simulink model "sm_car"  (R2025a)
settings: Solver=ode23t  StartTime=0.0  StopTime=400  MaxStep=0.4  RelTol=1e-3  AbsTol=1e-3  EnableMultiTasking=on
PreLoadFcn:
  | % Due to usability issue in Repeating Sequence block
  | warning('off','Simulink:Masking:Invalid');
  | 
  | % Eliminate unnecessary warnings in inactive variants
  | % Warnings generated only if you click through inactive variant
  | warning('off','MATLAB:nonExistentField');
  | warning('off','Simulink:Parameters:BlkParamUndefined');
PostLoadFcn:
  | set_param([bdroot '/Vehicle'],'popup_trailer','Off')
  | warning('off','sm:sli:setup:compile:LocalSolverNotSupported')
  | %sm_car_config_maneuver(bdroot,'WOT Braking');
  | sm_car_config_vehicle(bdroot,'false');
  | sm_car_config_logging(bdroot);
InitFcn:
  | sm_car_config_camera;
  | Vehicle = sm_car_vehcfg_checkConfig(Vehicle);
  | sm_car_check_tire_model(bdroot);
StartFcn:
  | tic;
StopFcn:
  | Elapsed_Sim_Time = toc;
  | % disp(['Elapsed Sim Time = ' num2str(Elapsed_Sim_Time)]);
undefined symbols (not defined in the file): Axle1D, AxleIn, Camera, Control, Driver, Free, Init, Maneuver, Pedal, RaceFix, RaceSpin, Scene, ShaftL1, ShaftL2, ShaftR1, ShaftR2, Soft, Stiff, Visual, X, xy_data_car_side, Y, Z
libraries: sm_lib x1546, nesl_utility x528, fl_lib x480, SimscapeFluids_lib x61, sdl_lib x49, simulink x29, ee_lib x7, simulink_extras x6, Linkage_Systems x4, Tire_1x2x x4, AntiRollBar_Systems x2, Linkage_Decoupled x2
(part 16 of 79)

== system sm_car/Controller/TrqVec 4Motor/Brake Control/ABS/Valve Control L2/Subsystem ==
  OnT : Inport
  Constant : Constant  Value=0
  Constant1 : Constant
  Demux : Demux  Outputs=9
  Multiport Switch : MultiPortSwitch  DataPortOrder=Zero-based contiguous  Inputs=11  zeroidx=on  SaturateOnIntegerOverflow=off  InputSameDT=off
  Pulse Generator : DiscretePulseGenerator  PulseType=Time based  Period=0.01  PulseWidth=[1 2 3 4 5 6 7 8 9]*10
  vSig : Outport  VectorParamsAs1DForOutWhenUnconnected=off
  wires:
  Multiport Switch/1 -> vSig/1
  Demux/9 -> Multiport Switch/11
  Demux/8 -> Multiport Switch/10
  Demux/7 -> Multiport Switch/9
  Demux/6 -> Multiport Switch/8
  Demux/5 -> Multiport Switch/7
  Demux/4 -> Multiport Switch/6
  Demux/3 -> Multiport Switch/5
  Demux/2 -> Multiport Switch/4
  Demux/1 -> Multiport Switch/3
  OnT/1 -> Multiport Switch/1
  Constant1/1 -> Multiport Switch/12
  Constant/1 -> Multiport Switch/2
  Pulse Generator/1 -> Demux/1

== system sm_car/Controller/TrqVec 4Motor/Brake Control/ABS/Valve Control L2/Subsystem1 ==
  OnT : Inport
  Constant : Constant  Value=0
  Constant1 : Constant
  Demux : Demux  Outputs=9
  Multiport Switch : MultiPortSwitch  DataPortOrder=Zero-based contiguous  Inputs=11  zeroidx=on  SaturateOnIntegerOverflow=off  InputSameDT=off
  Pulse Generator : DiscretePulseGenerator  PulseType=Time based  Period=0.01  PulseWidth=[1 2 3 4 5 6 7 8 9]*10
  vSig : Outport  VectorParamsAs1DForOutWhenUnconnected=off
  wires:
  Pulse Generator/1 -> Demux/1
  Constant/1 -> Multiport Switch/2
  Constant1/1 -> Multiport Switch/12
  OnT/1 -> Multiport Switch/1
  Demux/1 -> Multiport Switch/3
  Demux/2 -> Multiport Switch/4
  Demux/3 -> Multiport Switch/5
  Demux/4 -> Multiport Switch/6
  Demux/5 -> Multiport Switch/7
  Demux/6 -> Multiport Switch/8
  Demux/7 -> Multiport Switch/9
  Demux/8 -> Multiport Switch/10
  Demux/9 -> Multiport Switch/11
  Multiport Switch/1 -> vSig/1

== system sm_car/Controller/TrqVec 4Motor/Brake Control/ABS/Valve Control R1/Categorize Surface ==
  Mod State : Inport
  Apply Valve : Inport  Port=2
  Compare To Constant : simulink/Logic and Bit Operations/Compare To Constant  relop=<  const=4  OutDataTypeStr=boolean
  Compare To Constant1 : simulink/Logic and Bit Operations/Compare To Constant  relop===  const=2  OutDataTypeStr=boolean
  Count Apply Pulses : Subsystem  TreatAsAtomicUnit=on
  Terminator : Terminator
  Total Apply Pulses This Cycle : Subsystem  TreatAsAtomicUnit=on
  wires:
  Compare To Constant/1 -> Terminator/1  "Low Mu"
  Total Apply Pulses This Cycle/1(Total Pulses) -> Compare To Constant/1
  Compare To Constant1/1 -> Count Apply Pulses/1(In1)
  Mod State/1 -> Compare To Constant1/1, Total Apply Pulses This Cycle/Trigger  "Transition to Release"
  Apply Valve/1 -> Count Apply Pulses/Trigger
  Count Apply Pulses/1(Apply Pulses) -> Total Apply Pulses This Cycle/1(In1)

== system sm_car/Controller/TrqVec 4Motor/Brake Control/ABS/Valve Control R1/Code to Valves ==
  note: Release
  note: Hold
  note: Apply
  C : Inport
  Constant : Constant  Value=[0 0]
  Constant1 : Constant  Value=[0 1]
  Constant2 : Constant  Value=[1 0]
  Multiport Switch : MultiPortSwitch  DataPortOrder=Zero-based contiguous  zeroidx=on  SaturateOnIntegerOverflow=off  InputSameDT=off
  V : Outport  VectorParamsAs1DForOutWhenUnconnected=off
  wires:
  Multiport Switch/1 -> V/1
  C/1 -> Multiport Switch/1
  Constant2/1 -> Multiport Switch/4
  Constant1/1 -> Multiport Switch/3
  Constant/1 -> Multiport Switch/2

== system sm_car/Controller/TrqVec 4Motor/Brake Control/ABS/Valve Control R1/Subsystem ==
  OnT : Inport
  Constant : Constant  Value=0
  Constant1 : Constant
  Demux : Demux  Outputs=9
  Multiport Switch : MultiPortSwitch  DataPortOrder=Zero-based contiguous  Inputs=11  zeroidx=on  SaturateOnIntegerOverflow=off  InputSameDT=off
  Pulse Generator : DiscretePulseGenerator  PulseType=Time based  Period=0.01  PulseWidth=[1 2 3 4 5 6 7 8 9]*10
  vSig : Outport  VectorParamsAs1DForOutWhenUnconnected=off
  wires:
  Multiport Switch/1 -> vSig/1
  Demux/9 -> Multiport Switch/11
  Demux/8 -> Multiport Switch/10
  Demux/7 -> Multiport Switch/9
  Demux/6 -> Multiport Switch/8
  Demux/5 -> Multiport Switch/7
  Demux/4 -> Multiport Switch/6
  Demux/3 -> Multiport Switch/5
  Demux/2 -> Multiport Switch/4
  Demux/1 -> Multiport Switch/3
  OnT/1 -> Multiport Switch/1
  Constant1/1 -> Multiport Switch/12
  Constant/1 -> Multiport Switch/2
  Pulse Generator/1 -> Demux/1

== system sm_car/Controller/TrqVec 4Motor/Brake Control/ABS/Valve Control R1/Subsystem1 ==
  OnT : Inport
  Constant : Constant  Value=0
  Constant1 : Constant
  Demux : Demux  Outputs=9
  Multiport Switch : MultiPortSwitch  DataPortOrder=Zero-based contiguous  Inputs=11  zeroidx=on  SaturateOnIntegerOverflow=off  InputSameDT=off
  Pulse Generator : DiscretePulseGenerator  PulseType=Time based  Period=0.01  PulseWidth=[1 2 3 4 5 6 7 8 9]*10
  vSig : Outport  VectorParamsAs1DForOutWhenUnconnected=off
  wires:
  Pulse Generator/1 -> Demux/1
  Constant/1 -> Multiport Switch/2
  Constant1/1 -> Multiport Switch/12
  OnT/1 -> Multiport Switch/1
  Demux/1 -> Multiport Switch/3
  Demux/2 -> Multiport Switch/4
  Demux/3 -> Multiport Switch/5
  Demux/4 -> Multiport Switch/6
  Demux/5 -> Multiport Switch/7
  Demux/6 -> Multiport Switch/8
  Demux/7 -> Multiport Switch/9
  Demux/8 -> Multiport Switch/10
  Demux/9 -> Multiport Switch/11
  Multiport Switch/1 -> vSig/1

== system sm_car/Controller/TrqVec 4Motor/Brake Control/ABS/Valve Control R2/Categorize Surface ==
  Mod State : Inport
  Apply Valve : Inport  Port=2
  Compare To Constant : simulink/Logic and Bit Operations/Compare To Constant  relop=<  const=4  OutDataTypeStr=boolean
  Compare To Constant1 : simulink/Logic and Bit Operations/Compare To Constant  relop===  const=2  OutDataTypeStr=boolean
  Count Apply Pulses : Subsystem  TreatAsAtomicUnit=on
  Terminator : Terminator
  Total Apply Pulses This Cycle : Subsystem  TreatAsAtomicUnit=on
  wires:
  Compare To Constant/1 -> Terminator/1  "Low Mu"
  Total Apply Pulses This Cycle/1(Total Pulses) -> Compare To Constant/1
  Compare To Constant1/1 -> Count Apply Pulses/1(In1)
  Mod State/1 -> Compare To Constant1/1, Total Apply Pulses This Cycle/Trigger  "Transition to Release"
  Apply Valve/1 -> Count Apply Pulses/Trigger
  Count Apply Pulses/1(Apply Pulses) -> Total Apply Pulses This Cycle/1(In1)

== system sm_car/Controller/TrqVec 4Motor/Brake Control/ABS/Valve Control R2/Code to Valves ==
  note: Release
  note: Hold
  note: Apply
  C : Inport
  Constant : Constant  Value=[0 0]
  Constant1 : Constant  Value=[0 1]
  Constant2 : Constant  Value=[1 0]
  Multiport Switch : MultiPortSwitch  DataPortOrder=Zero-based contiguous  zeroidx=on  SaturateOnIntegerOverflow=off  InputSameDT=off
  V : Outport  VectorParamsAs1DForOutWhenUnconnected=off
  wires:
  Multiport Switch/1 -> V/1
  C/1 -> Multiport Switch/1
  Constant2/1 -> Multiport Switch/4
  Constant1/1 -> Multiport Switch/3
  Constant/1 -> Multiport Switch/2

== system sm_car/Controller/TrqVec 4Motor/Brake Control/ABS/Valve Control R2/Subsystem ==
  OnT : Inport
  Constant : Constant  Value=0
  Constant1 : Constant
  Demux : Demux  Outputs=9
  Multiport Switch : MultiPortSwitch  DataPortOrder=Zero-based contiguous  Inputs=11  zeroidx=on  SaturateOnIntegerOverflow=off  InputSameDT=off
  Pulse Generator : DiscretePulseGenerator  PulseType=Time based  Period=0.01  PulseWidth=[1 2 3 4 5 6 7 8 9]*10
  vSig : Outport  VectorParamsAs1DForOutWhenUnconnected=off
  wires:
  Multiport Switch/1 -> vSig/1
  Demux/9 -> Multiport Switch/11
  Demux/8 -> Multiport Switch/10
  Demux/7 -> Multiport Switch/9
  Demux/6 -> Multiport Switch/8
  Demux/5 -> Multiport Switch/7
  Demux/4 -> Multiport Switch/6
  Demux/3 -> Multiport Switch/5
  Demux/2 -> Multiport Switch/4
  Demux/1 -> Multiport Switch/3
  OnT/1 -> Multiport Switch/1
  Constant1/1 -> Multiport Switch/12
  Constant/1 -> Multiport Switch/2
  Pulse Generator/1 -> Demux/1

== system sm_car/Controller/TrqVec 4Motor/Brake Control/ABS/Valve Control R2/Subsystem1 ==
  OnT : Inport
  Constant : Constant  Value=0
  Constant1 : Constant
  Demux : Demux  Outputs=9
  Multiport Switch : MultiPortSwitch  DataPortOrder=Zero-based contiguous  Inputs=11  zeroidx=on  SaturateOnIntegerOverflow=off  InputSameDT=off
  Pulse Generator : DiscretePulseGenerator  PulseType=Time based  Period=0.01  PulseWidth=[1 2 3 4 5 6 7 8 9]*10
  vSig : Outport  VectorParamsAs1DForOutWhenUnconnected=off
  wires:
  Pulse Generator/1 -> Demux/1
  Constant/1 -> Multiport Switch/2
  Constant1/1 -> Multiport Switch/12
  OnT/1 -> Multiport Switch/1
  Demux/1 -> Multiport Switch/3
  Demux/2 -> Multiport Switch/4
  Demux/3 -> Multiport Switch/5
  Demux/4 -> Multiport Switch/6
  Demux/5 -> Multiport Switch/7
  Demux/6 -> Multiport Switch/8
  Demux/7 -> Multiport Switch/9
  Demux/8 -> Multiport Switch/10
  Demux/9 -> Multiport Switch/11
  Multiport Switch/1 -> vSig/1

== system sm_car/Controller/TrqVec 4Motor/Damper Control/Damper Control A1/Coefficient/Filter ==
  In : Inport
  Gain : Gain  Gain=1/b
  Integrator : Integrator  InitialCondition=x_initial*b
  Sum : Sum  Inputs=|+-  InputSameDT=on  SaturateOnIntegerOverflow=on  OutDataTypeStr=Inherit: Same as first input
  Out : Outport  VectorParamsAs1DForOutWhenUnconnected=off
  wires:
  Sum/1 -> Integrator/1
  In/1 -> Sum/1
  Integrator/1 -> Gain/1
  Gain/1 -> Sum/2, Out/1

== system sm_car/Controller/TrqVec 4Motor/Damper Control/Damper Control A1/Force/Filter ==
  In : Inport
  Gain : Gain  Gain=1/b
  Integrator : Integrator  InitialCondition=x_initial*b
  Sum : Sum  Inputs=|+-  InputSameDT=on  SaturateOnIntegerOverflow=on  OutDataTypeStr=Inherit: Same as first input
  Out : Outport  VectorParamsAs1DForOutWhenUnconnected=off
  wires:
  Sum/1 -> Integrator/1
  In/1 -> Sum/1
  Integrator/1 -> Gain/1
  Gain/1 -> Sum/2, Out/1

== system sm_car/Controller/TrqVec 4Motor/Damper Control/Damper Control A2/Coefficient/Filter ==
  In : Inport
  Gain : Gain  Gain=1/b
  Integrator : Integrator  InitialCondition=x_initial*b
  Sum : Sum  Inputs=|+-  InputSameDT=on  SaturateOnIntegerOverflow=on  OutDataTypeStr=Inherit: Same as first input
  Out : Outport  VectorParamsAs1DForOutWhenUnconnected=off
  wires:
  Sum/1 -> Integrator/1
  In/1 -> Sum/1
  Integrator/1 -> Gain/1
  Gain/1 -> Sum/2, Out/1

== system sm_car/Controller/TrqVec 4Motor/Damper Control/Damper Control A2/Force/Filter ==
  In : Inport
  Gain : Gain  Gain=1/b
  Integrator : Integrator  InitialCondition=x_initial*b
  Sum : Sum  Inputs=|+-  InputSameDT=on  SaturateOnIntegerOverflow=on  OutDataTypeStr=Inherit: Same as first input
  Out : Outport  VectorParamsAs1DForOutWhenUnconnected=off
  wires:
  Sum/1 -> Integrator/1
  In/1 -> Sum/1
  Integrator/1 -> Gain/1
  Gain/1 -> Sum/2, Out/1

== system sm_car/Vehicle/Vehicle/Chassis/Aero/Subsystem/Actuator dynamics ==
  In : Inport
  Gain : Gain  Gain=1/b
  Integrator : Integrator  InitialCondition=x_initial*b
  Sum : Sum  Inputs=|+-  InputSameDT=on  SaturateOnIntegerOverflow=on  OutDataTypeStr=Inherit: Same as first input
  Out : Outport  VectorParamsAs1DForOutWhenUnconnected=off
  wires:
  Sum/1 -> Integrator/1
  In/1 -> Sum/1
  Integrator/1 -> Gain/1
  Gain/1 -> Sum/2, Out/1

== system sm_car/Vehicle/Vehicle/Chassis/Body/Body Geometry/CAD FSAE Achilles ==
  Aero : Subsystem
  Body : Subsystem
  Rollbar : sm_lib/Body Elements/File Solid  ExtGeomFileName=FSAE_Rollbar.STL  UnitType=Custom  ExtGeomFileUnits=m  StepReaderType=HEX  ExportConvexHullGeometry=off  InertiaType=PointMass  BasedOnType=Density  Density=700.769  DensityUnits=kg/m^3  Mass=0  MassUnits=kg  CenterOfMass=[0.988684, 1.00464/1.8, 2.92072]  CenterOfMassUnits=m  MomentsOfInertia=[478.463, 518.088, 108.52]  MomentsOfInertiaUnits=kg*m^2  ProductsOfInertia=[-18.6469, 0.0347848, 0.00267861]  ProductsOfInertiaUnits=kg*m^2  GraphicType=FromGeometry  MarkerShape=Sphere  MarkerSize=10  GraphicVisPropType=SimpleVisualProperties  GraphicDiffuseColor=[0.6 0.6 0.6]  GraphicOpacity=1  GraphicSpecularColor=[0.5 0.5 0.5 1.0]  GraphicAmbientColor=[0.15 0.15 0.15 1.0]  GraphicEmissiveColor=[0.0 0.0 0.0 1.0]  GraphicShininess=75  DoExposeReferenceFrame=on  SerializedFrames=<Frames/>
  Seat : sm_lib/Body Elements/File Solid  ExtGeomFileName=FSAE_Seat.STL  UnitType=Custom  ExtGeomFileUnits=m  StepReaderType=HEX  ExportConvexHullGeometry=off  InertiaType=PointMass  BasedOnType=Density  Density=700.769  DensityUnits=kg/m^3  Mass=0  MassUnits=kg  CenterOfMass=[0.988684, 1.00464/1.8, 2.92072]  CenterOfMassUnits=m  MomentsOfInertia=[478.463, 518.088, 108.52]  MomentsOfInertiaUnits=kg*m^2  ProductsOfInertia=[-18.6469, 0.0347848, 0.00267861]  ProductsOfInertiaUnits=kg*m^2  GraphicType=FromGeometry  MarkerShape=Sphere  MarkerSize=10  GraphicVisPropType=SimpleVisualProperties  GraphicDiffuseColor=[0.2 0.2 0.2]  GraphicOpacity=1  GraphicSpecularColor=[0.5 0.5 0.5 1.0]  GraphicAmbientColor=[0.15 0.15 0.15 1.0]  GraphicEmissiveColor=[0.0 0.0 0.0 1.0]  GraphicShininess=75  DoExposeReferenceFrame=on  SerializedFrames=<Frames/>
  Transform CAD Offset : sm_lib/Frames and Transforms/Rigid Transform  RotationMethod=RotationSequence  FollAlignAxisA=+Y  BaseAlignAxisA=+Z  FollAlignAxisB=-X  BaseAlignAxisB=+Y  RotationStandardAxis=+Z  RotationAngle=0  RotationAngleUnits=deg  RotationArbitraryAxis=[0 0 1]  RotationSequenceAxes=FollowerAxes  RotationSequence=ZYX  RotationSequenceAngles=[body_orient(3) body_orient(2) body_orient(1)]  RotationSequenceAnglesUnits=rad  RotationMatrix=[1 0 0; 0 1 0; 0 0 1]  Quaternion=[1 0 0 0]  TranslationMethod=Cartesian  TranslationCartesianOffset=body_offset  TranslationCartesianOffsetUnits=m  TranslationStandardAxis=+Z  TranslationStandardOffset=0  TranslationStandardOffsetUnits=m  TranslationROffset=0  TranslationROffsetUnits=m  TranslationThetaOffset=0  TranslationThetaOffsetUnits=deg  TranslationZOffset=0  TranslationZOffsetUnits=m
  FA : PMIOPort  Side=Right
  P : PMIOPort  Port=2  Side=Left
  connections:
  Aero/RConn1 -- Transform CAD Offset/RConn1 -- Seat/RConn1 -- Body/LConn1 -- Rollbar/RConn1
  FA/RConn1 -- P/RConn1 -- Transform CAD Offset/LConn1

== system sm_car/Vehicle/Vehicle/Chassis/Body/Body Load/None ==
  FA : PMIOPort  Side=Left

== system sm_car/Vehicle/Vehicle/Chassis/Body/Body Sensor/Roll Pitch ==
  R : Inport
  Calculate aPitch : Subsystem
  Calculate aRoll : Subsystem
  "Flip sign for -x axis " : Gain  Gain=-1
  Select x axis : Selector  NumberOfDimensions=2  InputPortWidth=2  IndexOptions=Index vector (dialog),Index vector (dialog)  Indices=[1 2 3],1  OutputSizes=1,1
  Select y axis : Selector  NumberOfDimensions=2  InputPortWidth=2  IndexOptions=Index vector (dialog),Index vector (dialog)  Indices=[1 2 3],2  OutputSizes=1,1
  Transfer Fcn : TransferFcn  Numerator=[1 0]  Denominator=[0.01 1]
  Transfer Fcn1 : TransferFcn  Numerator=[1 0]  Denominator=[0.01 1]
  aRoll : Outport  VectorParamsAs1DForOutWhenUnconnected=off
  aPitch : Outport  Port=2  VectorParamsAs1DForOutWhenUnconnected=off
  nRoll : Outport  Port=3  VectorParamsAs1DForOutWhenUnconnected=off
  nPitch : Outport  Port=4  VectorParamsAs1DForOutWhenUnconnected=off
  wires:
  Calculate aPitch/1(Angle) -> "Flip sign for -x axis "/1
  Select x axis/1 -> Calculate aPitch/2(uvec)
  R/1 -> Select y axis/1, Select x axis/1
  Select y axis/1 -> Calculate aRoll/1(uvec)
  "Flip sign for -x axis "/1 -> aPitch/1, Transfer Fcn1/1
  Calculate aRoll/1(Angle) -> Transfer Fcn/1, aRoll/1, Calculate aPitch/1(Roll Angle)
  Transfer Fcn/1 -> nRoll/1
  Transfer Fcn1/1 -> nPitch/1

== system sm_car/Vehicle/Vehicle/Chassis/Body/Passenger FL/None ==
  Body Sensor Empty : Subsystem  mask{offset_body_sensor=Vehicle.Chassis.Body.sCG.Value}
      mask prompts: offset_body_sensor "Sensor Frame Offset [x y z] (m)"
  P : PMIOPort  Side=Left
  m : Outport  VectorParamsAs1DForOutWhenUnconnected=off
  wires:
  Body Sensor Empty/1(Body) -> m/1
  connections:
  Body Sensor Empty/LConn1 -- P/RConn1

== system sm_car/Vehicle/Vehicle/Chassis/Body/Passenger FR/None ==
  Body Sensor Empty : Subsystem  mask{offset_body_sensor=Vehicle.Chassis.Body.sCG.Value}
      mask prompts: offset_body_sensor "Sensor Frame Offset [x y z] (m)"
  P : PMIOPort  Side=Left
  m : Outport  VectorParamsAs1DForOutWhenUnconnected=off
  wires:
  Body Sensor Empty/1(Body) -> m/1
  connections:
  Body Sensor Empty/LConn1 -- P/RConn1

== system sm_car/Vehicle/Vehicle/Chassis/Body/Passenger RL/None ==
  Body Sensor Empty : Subsystem  mask{offset_body_sensor=Vehicle.Chassis.Body.sCG.Value}
      mask prompts: offset_body_sensor "Sensor Frame Offset [x y z] (m)"
  P : PMIOPort  Side=Left
  m : Outport  VectorParamsAs1DForOutWhenUnconnected=off
  wires:
  Body Sensor Empty/1(Body) -> m/1
  connections:
  Body Sensor Empty/LConn1 -- P/RConn1

== system sm_car/Vehicle/Vehicle/Chassis/Body/Passenger RR/None ==
  Body Sensor Empty : Subsystem  mask{offset_body_sensor=Vehicle.Chassis.Body.sCG.Value}
      mask prompts: offset_body_sensor "Sensor Frame Offset [x y z] (m)"
  P : PMIOPort  Side=Left
  m : Outport  VectorParamsAs1DForOutWhenUnconnected=off
  wires:
  Body Sensor Empty/1(Body) -> m/1
  connections:
  Body Sensor Empty/LConn1 -- P/RConn1

== system sm_car/Vehicle/Vehicle/Chassis/Damper/Decoupled/Damper A1 Heave ==
  "Ctrl " : Inport
  Force Endstop NL : Subsystem  VariantControl=Force_EndstopNL  mask(Variable Damping Force with Nonlinear Endstop){hp_dpr_top=Damper.Damping.sTop.Value, hp_dpr_bot=Damper.Damping.sBottom.Value, xEndstop=Damper.Endstop.xEndstop.Value, fEndstop=Damper.Endstop.fEndstop.Value}
      mask prompts: hp_dpr_top "HP Damper Top [xyz] (m)"; hp_dpr_bot "HP Damper Bottom [xyz] (m)"; xEndstop "Endstop Deformation Vector (m)"; fEndstop "Endstop Force Vector (m)"
      mask help: Variable damping force with a nonlinear endstop at top and bottom. The damping force is set using an input signal.
      mask init:
      | dam_x0 = norm(hp_dpr_top - hp_dpr_bot);
  Linear : Subsystem  VariantControl=Linear  mask(Linear Damper with Bumpstop){dam_b=Damper.Damping.d.Value, hp_dpr_top=Damper.Damping.sTop.Value, hp_dpr_bot=Damper.Damping.sBottom.Value, bs_lim_upper=Damper.Endstop.xMax.Value, bs_lim_lower=Damper.Endstop.xMin.Value, bs_k_upper=Damper.Endstop.KxMax.Value, bs_k_lower=Damper.Endstop.KxMin.Value, bs_b_upper=Damper.Endstop.dxMax.Value, bs_b_lower=Damper.Endstop.dxMin.Value, bs_region=Damper.Endstop.xTransition.Value}
      mask prompts: dam_b "Damper (N/(m/s))"; hp_dpr_top "HP Damper Top [xyz] (m)"; hp_dpr_bot "HP Damper Bottom [xyz] (m)"; bs_region "Transition Region (m)"
      mask help: Linear damper with bumpstop at top and bottom.
      mask init:
      | dam_x0 = norm(hp_dpr_top - hp_dpr_bot);
      mask TypeOptions dam_b: Damper/D
      mask DialogControl text_bumpstop_upper Prompt: Upper
      mask DialogControl text_bumpstop_lower Prompt: Lower
      mask DialogControl text_bumpstop_limit Prompt: Limit (m)
      mask DialogControl text_bumpstop_k Prompt: Stiffness (N/m)
      mask DialogControl text_bumpstop_b Prompt: Damping  (N/(m/s))
  None : Subsystem  VariantControl=None  mask(No Damper){}
      mask help: Sensor only
  Nonlinear : Subsystem  VariantControl=Nonlinear  mask(Nonlinear Damper with Bumpstop){velocity_vector=Damper.Damping.vDamper.Value, force_vector=Damper.Damping.fDamper.Value, hp_dpr_top=Damper.Damping.sTop.Value, hp_dpr_bot=Damper.Damping.sBottom.Value, bs_lim_upper=Damper.Endstop.xMax.Value, bs_lim_lower=Damper.Endstop.xMin.Value, bs_k_upper=Damper.Endstop.KxMax.Value, bs_k_lower=Damper.Endstop.KxMin.Value, bs_b_upper=Damper.Endstop.dxMax.Value, bs_b_lower=Damper.Endstop.dxMin.Value, bs_region=Damper.Endstop.xTransition.Value}
      mask prompts: velocity_vector "Velocity vector"; force_vector "Force vector"; hp_dpr_top "HP Damper Top [xyz] (m)"; hp_dpr_bot "HP Damper Bottom [xyz] (m)"; bs_region "Transition Region (m)"
      mask help: Damper with damping coefficient specified as a lookup table in parallel with a bumpstop.
      mask init:
      | dam_x0 = norm(hp_dpr_top - hp_dpr_bot);
      mask TypeOptions velocity_vector: Damper/velocity_vector
      mask TypeOptions force_vector: Damper/force_vector
      mask DialogControl text_bumpstop_upper Prompt: Upper
      mask DialogControl text_bumpstop_lower Prompt: Lower
      mask DialogControl text_bumpstop_limit Prompt: Limit (m)
      mask DialogControl text_bumpstop_k Prompt: Stiffness (N/m)
      mask DialogControl text_bumpstop_b Prompt: Damping  (N/(m/s))
  Nonlinear Endstop NL : Subsystem  VariantControl=Nonlinear_EndstopNL  mask(Nonlinear Damper with Nonlinear Bumpstop){velocity_vector=Damper.Damping.vDamper.Value, force_vector=Damper.Damping.fDamper.Value, hp_dpr_top=Damper.Damping.sTop.Value, hp_dpr_bot=Damper.Damping.sBottom.Value, xEndstop=Damper.Endstop.xEndstop.Value, fEndstop=Damper.Endstop.fEndstop.Value}
      mask prompts: velocity_vector "Velocity vector"; force_vector "Force vector"; hp_dpr_top "HP Damper Top [xyz] (m)"; hp_dpr_bot "HP Damper Bottom [xyz] (m)"; xEndstop "Endstop Deformation Vector (m)"; fEndstop "Endstop Force Vector (m)"
      mask help: Damper with damping coefficient specified as a lookup table in parallel with a nonlinear endstop at top and bottom.
      mask init:
      | dam_x0 = norm(hp_dpr_top - hp_dpr_bot);
      mask TypeOptions velocity_vector: Damper/velocity_vector
      mask TypeOptions force_vector: Damper/force_vector
      mask TypeOptions xEndstop: Bumpstop/deformation_vector
      mask TypeOptions fEndstop: Bumpstop/force_vector
  Variable : Subsystem  VariantControl=Variable  mask(Variable Damper with Endstop){hp_dpr_top=Damper.Damping.sTop.Value, hp_dpr_bot=Damper.Damping.sBottom.Value, bs_lim_upper=Damper.Endstop.xMax.Value, bs_lim_lower=Damper.Endstop.xMin.Value, bs_k_upper=Damper.Endstop.KxMax.Value, bs_k_lower=Damper.Endstop.KxMin.Value, bs_b_upper=Damper.Endstop.dxMax.Value, bs_b_lower=Damper.Endstop.dxMin.Value, bs_region=Damper.Endstop.xTransition.Value}
      mask prompts: hp_dpr_top "HP Damper Top [xyz] (m)"; hp_dpr_bot "HP Damper Bottom [xyz] (m)"; bs_region "Transition Region (m)"
      mask help: Variable damper with endstop at top and bottom. The damping coefficient is set using an input signal.
      mask init:
      | dam_x0 = norm(hp_dpr_top - hp_dpr_bot);
      mask DialogControl text_bumpstop_upper Prompt: Upper
      mask DialogControl text_bumpstop_lower Prompt: Lower
      mask DialogControl text_bumpstop_limit Prompt: Limit (m)
      mask DialogControl text_bumpstop_k Prompt: Stiffness (N/m)
      mask DialogControl text_bumpstop_b Prompt: Damping  (N/(m/s))
  Variable Endstop NL : Subsystem  VariantControl=Variable_EndstopNL  mask(Variable Damper with Nonlinear Endstop){hp_dpr_top=Damper.Damping.sTop.Value, hp_dpr_bot=Damper.Damping.sBottom.Value, xEndstop=Damper.Endstop.xEndstop.Value, fEndstop=Damper.Endstop.fEndstop.Value}
      mask prompts: hp_dpr_top "HP Damper Top [xyz] (m)"; hp_dpr_bot "HP Damper Bottom [xyz] (m)"; xEndstop "Endstop Deformation Vector (m)"; fEndstop "Endstop Force Vector (m)"
      mask help: Variable damper with nonlinear endstop at top and bottom. The damping coefficient is set using an input signal.
      mask init:
      | dam_x0 = norm(hp_dpr_top - hp_dpr_bot);
  " R" : PMIOPort  Side=Left
  " C" : PMIOPort  Port=2  Side=Right
  " meas" : Outport  VectorParamsAs1DForOutWhenUnconnected=off

== system sm_car/Vehicle/Vehicle/Chassis/Damper/Decoupled/Damper A1 Roll ==
  "Ctrl " : Inport
  Force Endstop NL : Subsystem  VariantControl=Force_EndstopNL  mask(Variable Damping Force with Nonlinear Endstop){hp_dpr_top=Damper.Damping.sTop.Value, hp_dpr_bot=Damper.Damping.sBottom.Value, xEndstop=Damper.Endstop.xEndstop.Value, fEndstop=Damper.Endstop.fEndstop.Value}
      mask prompts: hp_dpr_top "HP Damper Top [xyz] (m)"; hp_dpr_bot "HP Damper Bottom [xyz] (m)"; xEndstop "Endstop Deformation Vector (m)"; fEndstop "Endstop Force Vector (m)"
      mask help: Variable damping force with a nonlinear endstop at top and bottom. The damping force is set using an input signal.
      mask init:
      | dam_x0 = norm(hp_dpr_top - hp_dpr_bot);
  Linear : Subsystem  VariantControl=Linear  mask(Linear Damper with Bumpstop){dam_b=Damper.Damping.d.Value, hp_dpr_top=Damper.Damping.sTop.Value, hp_dpr_bot=Damper.Damping.sBottom.Value, bs_lim_upper=Damper.Endstop.xMax.Value, bs_lim_lower=Damper.Endstop.xMin.Value, bs_k_upper=Damper.Endstop.KxMax.Value, bs_k_lower=Damper.Endstop.KxMin.Value, bs_b_upper=Damper.Endstop.dxMax.Value, bs_b_lower=Damper.Endstop.dxMin.Value, bs_region=Damper.Endstop.xTransition.Value}
      mask prompts: dam_b "Damper (N/(m/s))"; hp_dpr_top "HP Damper Top [xyz] (m)"; hp_dpr_bot "HP Damper Bottom [xyz] (m)"; bs_region "Transition Region (m)"
      mask help: Linear damper with bumpstop at top and bottom.
      mask init:
      | dam_x0 = norm(hp_dpr_top - hp_dpr_bot);
      mask TypeOptions dam_b: Damper/D
      mask DialogControl text_bumpstop_upper Prompt: Upper
      mask DialogControl text_bumpstop_lower Prompt: Lower
      mask DialogControl text_bumpstop_limit Prompt: Limit (m)
      mask DialogControl text_bumpstop_k Prompt: Stiffness (N/m)
      mask DialogControl text_bumpstop_b Prompt: Damping  (N/(m/s))
  None : Subsystem  VariantControl=None  mask(No Damper){}
      mask help: Sensor only
  Nonlinear : Subsystem  VariantControl=Nonlinear  mask(Nonlinear Damper with Bumpstop){velocity_vector=Damper.Damping.vDamper.Value, force_vector=Damper.Damping.fDamper.Value, hp_dpr_top=Damper.Damping.sTop.Value, hp_dpr_bot=Damper.Damping.sBottom.Value, bs_lim_upper=Damper.Endstop.xMax.Value, bs_lim_lower=Damper.Endstop.xMin.Value, bs_k_upper=Damper.Endstop.KxMax.Value, bs_k_lower=Damper.Endstop.KxMin.Value, bs_b_upper=Damper.Endstop.dxMax.Value, bs_b_lower=Damper.Endstop.dxMin.Value, bs_region=Damper.Endstop.xTransition.Value}
      mask prompts: velocity_vector "Velocity vector"; force_vector "Force vector"; hp_dpr_top "HP Damper Top [xyz] (m)"; hp_dpr_bot "HP Damper Bottom [xyz] (m)"; bs_region "Transition Region (m)"
      mask help: Damper with damping coefficient specified as a lookup table in parallel with a bumpstop.
      mask init:
      | dam_x0 = norm(hp_dpr_top - hp_dpr_bot);
      mask TypeOptions velocity_vector: Damper/velocity_vector
      mask TypeOptions force_vector: Damper/force_vector
      mask DialogControl text_bumpstop_upper Prompt: Upper
      mask DialogControl text_bumpstop_lower Prompt: Lower
      mask DialogControl text_bumpstop_limit Prompt: Limit (m)
      mask DialogControl text_bumpstop_k Prompt: Stiffness (N/m)
      mask DialogControl text_bumpstop_b Prompt: Damping  (N/(m/s))
  Nonlinear Endstop NL : Subsystem  VariantControl=Nonlinear_EndstopNL  mask(Nonlinear Damper with Nonlinear Bumpstop){velocity_vector=Damper.Damping.vDamper.Value, force_vector=Damper.Damping.fDamper.Value, hp_dpr_top=Damper.Damping.sTop.Value, hp_dpr_bot=Damper.Damping.sBottom.Value, xEndstop=Damper.Endstop.xEndstop.Value, fEndstop=Damper.Endstop.fEndstop.Value}
      mask prompts: velocity_vector "Velocity vector"; force_vector "Force vector"; hp_dpr_top "HP Damper Top [xyz] (m)"; hp_dpr_bot "HP Damper Bottom [xyz] (m)"; xEndstop "Endstop Deformation Vector (m)"; fEndstop "Endstop Force Vector (m)"
      mask help: Damper with damping coefficient specified as a lookup table in parallel with a nonlinear endstop at top and bottom.
      mask init:
      | dam_x0 = norm(hp_dpr_top - hp_dpr_bot);
      mask TypeOptions velocity_vector: Damper/velocity_vector
      mask TypeOptions force_vector: Damper/force_vector
      mask TypeOptions xEndstop: Bumpstop/deformation_vector
      mask TypeOptions fEndstop: Bumpstop/force_vector
  Variable : Subsystem  VariantControl=Variable  mask(Variable Damper with Endstop){hp_dpr_top=Damper.Damping.sTop.Value, hp_dpr_bot=Damper.Damping.sBottom.Value, bs_lim_upper=Damper.Endstop.xMax.Value, bs_lim_lower=Damper.Endstop.xMin.Value, bs_k_upper=Damper.Endstop.KxMax.Value, bs_k_lower=Damper.Endstop.KxMin.Value, bs_b_upper=Damper.Endstop.dxMax.Value, bs_b_lower=Damper.Endstop.dxMin.Value, bs_region=Damper.Endstop.xTransition.Value}
      mask prompts: hp_dpr_top "HP Damper Top [xyz] (m)"; hp_dpr_bot "HP Damper Bottom [xyz] (m)"; bs_region "Transition Region (m)"
      mask help: Variable damper with endstop at top and bottom. The damping coefficient is set using an input signal.
      mask init:
      | dam_x0 = norm(hp_dpr_top - hp_dpr_bot);
      mask DialogControl text_bumpstop_upper Prompt: Upper
      mask DialogControl text_bumpstop_lower Prompt: Lower
      mask DialogControl text_bumpstop_limit Prompt: Limit (m)
      mask DialogControl text_bumpstop_k Prompt: Stiffness (N/m)
      mask DialogControl text_bumpstop_b Prompt: Damping  (N/(m/s))
  Variable Endstop NL : Subsystem  VariantControl=Variable_EndstopNL  mask(Variable Damper with Nonlinear Endstop){hp_dpr_top=Damper.Damping.sTop.Value, hp_dpr_bot=Damper.Damping.sBottom.Value, xEndstop=Damper.Endstop.xEndstop.Value, fEndstop=Damper.Endstop.fEndstop.Value}
      mask prompts: hp_dpr_top "HP Damper Top [xyz] (m)"; hp_dpr_bot "HP Damper Bottom [xyz] (m)"; xEndstop "Endstop Deformation Vector (m)"; fEndstop "Endstop Force Vector (m)"
      mask help: Variable damper with nonlinear endstop at top and bottom. The damping coefficient is set using an input signal.
      mask init:
      | dam_x0 = norm(hp_dpr_top - hp_dpr_bot);
  " R" : PMIOPort  Side=Left
  " C" : PMIOPort  Port=2  Side=Right
  " meas" : Outport  VectorParamsAs1DForOutWhenUnconnected=off

== system sm_car/Vehicle/Vehicle/Chassis/Damper/Decoupled/Damper A2 Heave ==
  "Ctrl " : Inport
  Force Endstop NL : Subsystem  VariantControl=Force_EndstopNL  mask(Variable Damping Force with Nonlinear Endstop){hp_dpr_top=Damper.Damping.sTop.Value, hp_dpr_bot=Damper.Damping.sBottom.Value, xEndstop=Damper.Endstop.xEndstop.Value, fEndstop=Damper.Endstop.fEndstop.Value}
      mask prompts: hp_dpr_top "HP Damper Top [xyz] (m)"; hp_dpr_bot "HP Damper Bottom [xyz] (m)"; xEndstop "Endstop Deformation Vector (m)"; fEndstop "Endstop Force Vector (m)"
      mask help: Variable damping force with a nonlinear endstop at top and bottom. The damping force is set using an input signal.
      mask init:
      | dam_x0 = norm(hp_dpr_top - hp_dpr_bot);
  Linear : Subsystem  VariantControl=Linear  mask(Linear Damper with Bumpstop){dam_b=Damper.Damping.d.Value, hp_dpr_top=Damper.Damping.sTop.Value, hp_dpr_bot=Damper.Damping.sBottom.Value, bs_lim_upper=Damper.Endstop.xMax.Value, bs_lim_lower=Damper.Endstop.xMin.Value, bs_k_upper=Damper.Endstop.KxMax.Value, bs_k_lower=Damper.Endstop.KxMin.Value, bs_b_upper=Damper.Endstop.dxMax.Value, bs_b_lower=Damper.Endstop.dxMin.Value, bs_region=Damper.Endstop.xTransition.Value}
      mask prompts: dam_b "Damper (N/(m/s))"; hp_dpr_top "HP Damper Top [xyz] (m)"; hp_dpr_bot "HP Damper Bottom [xyz] (m)"; bs_region "Transition Region (m)"
      mask help: Linear damper with bumpstop at top and bottom.
      mask init:
      | dam_x0 = norm(hp_dpr_top - hp_dpr_bot);
      mask TypeOptions dam_b: Damper/D
      mask DialogControl text_bumpstop_upper Prompt: Upper
      mask DialogControl text_bumpstop_lower Prompt: Lower
      mask DialogControl text_bumpstop_limit Prompt: Limit (m)
      mask DialogControl text_bumpstop_k Prompt: Stiffness (N/m)
      mask DialogControl text_bumpstop_b Prompt: Damping  (N/(m/s))
  None : Subsystem  VariantControl=None  mask(No Damper){}
      mask help: Sensor only
  Nonlinear : Subsystem  VariantControl=Nonlinear  mask(Nonlinear Damper with Bumpstop){velocity_vector=Damper.Damping.vDamper.Value, force_vector=Damper.Damping.fDamper.Value, hp_dpr_top=Damper.Damping.sTop.Value, hp_dpr_bot=Damper.Damping.sBottom.Value, bs_lim_upper=Damper.Endstop.xMax.Value, bs_lim_lower=Damper.Endstop.xMin.Value, bs_k_upper=Damper.Endstop.KxMax.Value, bs_k_lower=Damper.Endstop.KxMin.Value, bs_b_upper=Damper.Endstop.dxMax.Value, bs_b_lower=Damper.Endstop.dxMin.Value, bs_region=Damper.Endstop.xTransition.Value}
      mask prompts: velocity_vector "Velocity vector"; force_vector "Force vector"; hp_dpr_top "HP Damper Top [xyz] (m)"; hp_dpr_bot "HP Damper Bottom [xyz] (m)"; bs_region "Transition Region (m)"
      mask help: Damper with damping coefficient specified as a lookup table in parallel with a bumpstop.
      mask init:
      | dam_x0 = norm(hp_dpr_top - hp_dpr_bot);
      mask TypeOptions velocity_vector: Damper/velocity_vector
      mask TypeOptions force_vector: Damper/force_vector
      mask DialogControl text_bumpstop_upper Prompt: Upper
      mask DialogControl text_bumpstop_lower Prompt: Lower
      mask DialogControl text_bumpstop_limit Prompt: Limit (m)
      mask DialogControl text_bumpstop_k Prompt: Stiffness (N/m)
      mask DialogControl text_bumpstop_b Prompt: Damping  (N/(m/s))
  Nonlinear Endstop NL : Subsystem  VariantControl=Nonlinear_EndstopNL  mask(Nonlinear Damper with Nonlinear Bumpstop){velocity_vector=Damper.Damping.vDamper.Value, force_vector=Damper.Damping.fDamper.Value, hp_dpr_top=Damper.Damping.sTop.Value, hp_dpr_bot=Damper.Damping.sBottom.Value, xEndstop=Damper.Endstop.xEndstop.Value, fEndstop=Damper.Endstop.fEndstop.Value}
      mask prompts: velocity_vector "Velocity vector"; force_vector "Force vector"; hp_dpr_top "HP Damper Top [xyz] (m)"; hp_dpr_bot "HP Damper Bottom [xyz] (m)"; xEndstop "Endstop Deformation Vector (m)"; fEndstop "Endstop Force Vector (m)"
      mask help: Damper with damping coefficient specified as a lookup table in parallel with a nonlinear endstop at top and bottom.
      mask init:
      | dam_x0 = norm(hp_dpr_top - hp_dpr_bot);
      mask TypeOptions velocity_vector: Damper/velocity_vector
      mask TypeOptions force_vector: Damper/force_vector
      mask TypeOptions xEndstop: Bumpstop/deformation_vector
      mask TypeOptions fEndstop: Bumpstop/force_vector
  Variable : Subsystem  VariantControl=Variable  mask(Variable Damper with Endstop){hp_dpr_top=Damper.Damping.sTop.Value, hp_dpr_bot=Damper.Damping.sBottom.Value, bs_lim_upper=Damper.Endstop.xMax.Value, bs_lim_lower=Damper.Endstop.xMin.Value, bs_k_upper=Damper.Endstop.KxMax.Value, bs_k_lower=Damper.Endstop.KxMin.Value, bs_b_upper=Damper.Endstop.dxMax.Value, bs_b_lower=Damper.Endstop.dxMin.Value, bs_region=Damper.Endstop.xTransition.Value}
      mask prompts: hp_dpr_top "HP Damper Top [xyz] (m)"; hp_dpr_bot "HP Damper Bottom [xyz] (m)"; bs_region "Transition Region (m)"
      mask help: Variable damper with endstop at top and bottom. The damping coefficient is set using an input signal.
      mask init:
      | dam_x0 = norm(hp_dpr_top - hp_dpr_bot);
      mask DialogControl text_bumpstop_upper Prompt: Upper
      mask DialogControl text_bumpstop_lower Prompt: Lower
      mask DialogControl text_bumpstop_limit Prompt: Limit (m)
      mask DialogControl text_bumpstop_k Prompt: Stiffness (N/m)
      mask DialogControl text_bumpstop_b Prompt: Damping  (N/(m/s))
  Variable Endstop NL : Subsystem  VariantControl=Variable_EndstopNL  mask(Variable Damper with Nonlinear Endstop){hp_dpr_top=Damper.Damping.sTop.Value, hp_dpr_bot=Damper.Damping.sBottom.Value, xEndstop=Damper.Endstop.xEndstop.Value, fEndstop=Damper.Endstop.fEndstop.Value}
      mask prompts: hp_dpr_top "HP Damper Top [xyz] (m)"; hp_dpr_bot "HP Damper Bottom [xyz] (m)"; xEndstop "Endstop Deformation Vector (m)"; fEndstop "Endstop Force Vector (m)"
      mask help: Variable damper with nonlinear endstop at top and bottom. The damping coefficient is set using an input signal.
      mask init:
      | dam_x0 = norm(hp_dpr_top - hp_dpr_bot);
  " R" : PMIOPort  Side=Left
  " C" : PMIOPort  Port=2  Side=Right
  " meas" : Outport  VectorParamsAs1DForOutWhenUnconnected=off

== system sm_car/Vehicle/Vehicle/Chassis/Damper/Decoupled/Damper A2 Roll ==
  "Ctrl " : Inport
  Force Endstop NL : Subsystem  VariantControl=Force_EndstopNL  mask(Variable Damping Force with Nonlinear Endstop){hp_dpr_top=Damper.Damping.sTop.Value, hp_dpr_bot=Damper.Damping.sBottom.Value, xEndstop=Damper.Endstop.xEndstop.Value, fEndstop=Damper.Endstop.fEndstop.Value}
      mask prompts: hp_dpr_top "HP Damper Top [xyz] (m)"; hp_dpr_bot "HP Damper Bottom [xyz] (m)"; xEndstop "Endstop Deformation Vector (m)"; fEndstop "Endstop Force Vector (m)"
      mask help: Variable damping force with a nonlinear endstop at top and bottom. The damping force is set using an input signal.
      mask init:
      | dam_x0 = norm(hp_dpr_top - hp_dpr_bot);
  Linear : Subsystem  VariantControl=Linear  mask(Linear Damper with Bumpstop){dam_b=Damper.Damping.d.Value, hp_dpr_top=Damper.Damping.sTop.Value, hp_dpr_bot=Damper.Damping.sBottom.Value, bs_lim_upper=Damper.Endstop.xMax.Value, bs_lim_lower=Damper.Endstop.xMin.Value, bs_k_upper=Damper.Endstop.KxMax.Value, bs_k_lower=Damper.Endstop.KxMin.Value, bs_b_upper=Damper.Endstop.dxMax.Value, bs_b_lower=Damper.Endstop.dxMin.Value, bs_region=Damper.Endstop.xTransition.Value}
      mask prompts: dam_b "Damper (N/(m/s))"; hp_dpr_top "HP Damper Top [xyz] (m)"; hp_dpr_bot "HP Damper Bottom [xyz] (m)"; bs_region "Transition Region (m)"
      mask help: Linear damper with bumpstop at top and bottom.
      mask init:
      | dam_x0 = norm(hp_dpr_top - hp_dpr_bot);
      mask TypeOptions dam_b: Damper/D
      mask DialogControl text_bumpstop_upper Prompt: Upper
      mask DialogControl text_bumpstop_lower Prompt: Lower
      mask DialogControl text_bumpstop_limit Prompt: Limit (m)
      mask DialogControl text_bumpstop_k Prompt: Stiffness (N/m)
      mask DialogControl text_bumpstop_b Prompt: Damping  (N/(m/s))
  None : Subsystem  VariantControl=None  mask(No Damper){}
      mask help: Sensor only
  Nonlinear : Subsystem  VariantControl=Nonlinear  mask(Nonlinear Damper with Bumpstop){velocity_vector=Damper.Damping.vDamper.Value, force_vector=Damper.Damping.fDamper.Value, hp_dpr_top=Damper.Damping.sTop.Value, hp_dpr_bot=Damper.Damping.sBottom.Value, bs_lim_upper=Damper.Endstop.xMax.Value, bs_lim_lower=Damper.Endstop.xMin.Value, bs_k_upper=Damper.Endstop.KxMax.Value, bs_k_lower=Damper.Endstop.KxMin.Value, bs_b_upper=Damper.Endstop.dxMax.Value, bs_b_lower=Damper.Endstop.dxMin.Value, bs_region=Damper.Endstop.xTransition.Value}
      mask prompts: velocity_vector "Velocity vector"; force_vector "Force vector"; hp_dpr_top "HP Damper Top [xyz] (m)"; hp_dpr_bot "HP Damper Bottom [xyz] (m)"; bs_region "Transition Region (m)"
      mask help: Damper with damping coefficient specified as a lookup table in parallel with a bumpstop.
      mask init:
      | dam_x0 = norm(hp_dpr_top - hp_dpr_bot);
      mask TypeOptions velocity_vector: Damper/velocity_vector
      mask TypeOptions force_vector: Damper/force_vector
      mask DialogControl text_bumpstop_upper Prompt: Upper
      mask DialogControl text_bumpstop_lower Prompt: Lower
      mask DialogControl text_bumpstop_limit Prompt: Limit (m)
      mask DialogControl text_bumpstop_k Prompt: Stiffness (N/m)
      mask DialogControl text_bumpstop_b Prompt: Damping  (N/(m/s))
  Nonlinear Endstop NL : Subsystem  VariantControl=Nonlinear_EndstopNL  mask(Nonlinear Damper with Nonlinear Bumpstop){velocity_vector=Damper.Damping.vDamper.Value, force_vector=Damper.Damping.fDamper.Value, hp_dpr_top=Damper.Damping.sTop.Value, hp_dpr_bot=Damper.Damping.sBottom.Value, xEndstop=Damper.Endstop.xEndstop.Value, fEndstop=Damper.Endstop.fEndstop.Value}
      mask prompts: velocity_vector "Velocity vector"; force_vector "Force vector"; hp_dpr_top "HP Damper Top [xyz] (m)"; hp_dpr_bot "HP Damper Bottom [xyz] (m)"; xEndstop "Endstop Deformation Vector (m)"; fEndstop "Endstop Force Vector (m)"
      mask help: Damper with damping coefficient specified as a lookup table in parallel with a nonlinear endstop at top and bottom.
      mask init:
      | dam_x0 = norm(hp_dpr_top - hp_dpr_bot);
      mask TypeOptions velocity_vector: Damper/velocity_vector
      mask TypeOptions force_vector: Damper/force_vector
      mask TypeOptions xEndstop: Bumpstop/deformation_vector
      mask TypeOptions fEndstop: Bumpstop/force_vector
  Variable : Subsystem  VariantControl=Variable  mask(Variable Damper with Endstop){hp_dpr_top=Damper.Damping.sTop.Value, hp_dpr_bot=Damper.Damping.sBottom.Value, bs_lim_upper=Damper.Endstop.xMax.Value, bs_lim_lower=Damper.Endstop.xMin.Value, bs_k_upper=Damper.Endstop.KxMax.Value, bs_k_lower=Damper.Endstop.KxMin.Value, bs_b_upper=Damper.Endstop.dxMax.Value, bs_b_lower=Damper.Endstop.dxMin.Value, bs_region=Damper.Endstop.xTransition.Value}
      mask prompts: hp_dpr_top "HP Damper Top [xyz] (m)"; hp_dpr_bot "HP Damper Bottom [xyz] (m)"; bs_region "Transition Region (m)"
      mask help: Variable damper with endstop at top and bottom. The damping coefficient is set using an input signal.
      mask init:
      | dam_x0 = norm(hp_dpr_top - hp_dpr_bot);
      mask DialogControl text_bumpstop_upper Prompt: Upper
      mask DialogControl text_bumpstop_lower Prompt: Lower
      mask DialogControl text_bumpstop_limit Prompt: Limit (m)
      mask DialogControl text_bumpstop_k Prompt: Stiffness (N/m)
      mask DialogControl text_bumpstop_b Prompt: Damping  (N/(m/s))
  Variable Endstop NL : Subsystem  VariantControl=Variable_EndstopNL  mask(Variable Damper with Nonlinear Endstop){hp_dpr_top=Damper.Damping.sTop.Value, hp_dpr_bot=Damper.Damping.sBottom.Value, xEndstop=Damper.Endstop.xEndstop.Value, fEndstop=Damper.Endstop.fEndstop.Value}
      mask prompts: hp_dpr_top "HP Damper Top [xyz] (m)"; hp_dpr_bot "HP Damper Bottom [xyz] (m)"; xEndstop "Endstop Deformation Vector (m)"; fEndstop "Endstop Force Vector (m)"
      mask help: Variable damper with nonlinear endstop at top and bottom. The damping coefficient is set using an input signal.
      mask init:
      | dam_x0 = norm(hp_dpr_top - hp_dpr_bot);
  " R" : PMIOPort  Side=Left
  " C" : PMIOPort  Port=2  Side=Right
  " meas" : Outport  VectorParamsAs1DForOutWhenUnconnected=off

== system sm_car/Vehicle/Vehicle/Chassis/Damper/Independent/Damper L1 ==
  "Ctrl " : Inport
  Linear : Subsystem  VariantControl=Linear  mask(Linear Damper with Bumpstop){dam_b=Damper.Damping.d.Value, hp_dpr_top=Damper.Damping.sTop.Value, hp_dpr_bot=Damper.Damping.sBottom.Value, bs_lim_upper=Damper.Endstop.xMax.Value, bs_lim_lower=Damper.Endstop.xMin.Value, bs_k_upper=Damper.Endstop.KxMax.Value, bs_k_lower=Damper.Endstop.KxMin.Value, bs_b_upper=Damper.Endstop.dxMax.Value, bs_b_lower=Damper.Endstop.dxMin.Value, bs_region=Damper.Endstop.xTransition.Value}
      mask prompts: dam_b "Damper (N/(m/s))"; hp_dpr_top "HP Damper Top [xyz] (m)"; hp_dpr_bot "HP Damper Bottom [xyz] (m)"; bs_region "Transition Region (m)"
      mask help: Linear damper with bumpstop at top and bottom.
      mask init:
      | dam_x0 = norm(hp_dpr_top - hp_dpr_bot);
      mask TypeOptions dam_b: Damper/D
      mask DialogControl text_bumpstop_upper Prompt: Upper
      mask DialogControl text_bumpstop_lower Prompt: Lower
      mask DialogControl text_bumpstop_limit Prompt: Limit (m)
      mask DialogControl text_bumpstop_k Prompt: Stiffness (N/m)
      mask DialogControl text_bumpstop_b Prompt: Damping  (N/(m/s))
  " R" : PMIOPort  Side=Left
  " C" : PMIOPort  Port=2  Side=Right
  " meas" : Outport  VectorParamsAs1DForOutWhenUnconnected=off

== system sm_car/Vehicle/Vehicle/Chassis/Damper/Independent/Damper L2 ==
  "Ctrl " : Inport
  Linear : Subsystem  VariantControl=Linear  mask(Linear Damper with Bumpstop){dam_b=Damper.Damping.d.Value, hp_dpr_top=Damper.Damping.sTop.Value, hp_dpr_bot=Damper.Damping.sBottom.Value, bs_lim_upper=Damper.Endstop.xMax.Value, bs_lim_lower=Damper.Endstop.xMin.Value, bs_k_upper=Damper.Endstop.KxMax.Value, bs_k_lower=Damper.Endstop.KxMin.Value, bs_b_upper=Damper.Endstop.dxMax.Value, bs_b_lower=Damper.Endstop.dxMin.Value, bs_region=Damper.Endstop.xTransition.Value}
      mask prompts: dam_b "Damper (N/(m/s))"; hp_dpr_top "HP Damper Top [xyz] (m)"; hp_dpr_bot "HP Damper Bottom [xyz] (m)"; bs_region "Transition Region (m)"
      mask help: Linear damper with bumpstop at top and bottom.
      mask init:
      | dam_x0 = norm(hp_dpr_top - hp_dpr_bot);
      mask TypeOptions dam_b: Damper/D
      mask DialogControl text_bumpstop_upper Prompt: Upper
      mask DialogControl text_bumpstop_lower Prompt: Lower
      mask DialogControl text_bumpstop_limit Prompt: Limit (m)
      mask DialogControl text_bumpstop_k Prompt: Stiffness (N/m)
      mask DialogControl text_bumpstop_b Prompt: Damping  (N/(m/s))
  " R" : PMIOPort  Side=Left
  " C" : PMIOPort  Port=2  Side=Right
  " meas" : Outport  VectorParamsAs1DForOutWhenUnconnected=off

== system sm_car/Vehicle/Vehicle/Chassis/Damper/Independent/Damper R1 ==
  "Ctrl " : Inport
  Linear : Subsystem  VariantControl=Linear  mask(Linear Damper with Bumpstop){dam_b=Damper.Damping.d.Value, hp_dpr_top=Damper.Damping.sTop.Value, hp_dpr_bot=Damper.Damping.sBottom.Value, bs_lim_upper=Damper.Endstop.xMax.Value, bs_lim_lower=Damper.Endstop.xMin.Value, bs_k_upper=Damper.Endstop.KxMax.Value, bs_k_lower=Damper.Endstop.KxMin.Value, bs_b_upper=Damper.Endstop.dxMax.Value, bs_b_lower=Damper.Endstop.dxMin.Value, bs_region=Damper.Endstop.xTransition.Value}
      mask prompts: dam_b "Damper (N/(m/s))"; hp_dpr_top "HP Damper Top [xyz] (m)"; hp_dpr_bot "HP Damper Bottom [xyz] (m)"; bs_region "Transition Region (m)"
      mask help: Linear damper with bumpstop at top and bottom.
      mask init:
      | dam_x0 = norm(hp_dpr_top - hp_dpr_bot);
      mask TypeOptions dam_b: Damper/D
      mask DialogControl text_bumpstop_upper Prompt: Upper
      mask DialogControl text_bumpstop_lower Prompt: Lower
      mask DialogControl text_bumpstop_limit Prompt: Limit (m)
      mask DialogControl text_bumpstop_k Prompt: Stiffness (N/m)
      mask DialogControl text_bumpstop_b Prompt: Damping  (N/(m/s))
  " R" : PMIOPort  Side=Left
  " C" : PMIOPort  Port=2  Side=Right
  " meas" : Outport  VectorParamsAs1DForOutWhenUnconnected=off

== system sm_car/Vehicle/Vehicle/Chassis/Damper/Independent/Damper R2 ==
  "Ctrl " : Inport
  Linear : Subsystem  VariantControl=Linear  mask(Linear Damper with Bumpstop){dam_b=Damper.Damping.d.Value, hp_dpr_top=Damper.Damping.sTop.Value, hp_dpr_bot=Damper.Damping.sBottom.Value, bs_lim_upper=Damper.Endstop.xMax.Value, bs_lim_lower=Damper.Endstop.xMin.Value, bs_k_upper=Damper.Endstop.KxMax.Value, bs_k_lower=Damper.Endstop.KxMin.Value, bs_b_upper=Damper.Endstop.dxMax.Value, bs_b_lower=Damper.Endstop.dxMin.Value, bs_region=Damper.Endstop.xTransition.Value}
      mask prompts: dam_b "Damper (N/(m/s))"; hp_dpr_top "HP Damper Top [xyz] (m)"; hp_dpr_bot "HP Damper Bottom [xyz] (m)"; bs_region "Transition Region (m)"
      mask help: Linear damper with bumpstop at top and bottom.
      mask init:
      | dam_x0 = norm(hp_dpr_top - hp_dpr_bot);
      mask TypeOptions dam_b: Damper/D
      mask DialogControl text_bumpstop_upper Prompt: Upper
      mask DialogControl text_bumpstop_lower Prompt: Lower
      mask DialogControl text_bumpstop_limit Prompt: Limit (m)
      mask DialogControl text_bumpstop_k Prompt: Stiffness (N/m)
      mask DialogControl text_bumpstop_b Prompt: Damping  (N/(m/s))
  " R" : PMIOPort  Side=Left
  " C" : PMIOPort  Port=2  Side=Right
  " meas" : Outport  VectorParamsAs1DForOutWhenUnconnected=off
